simulink model "SMXQ6_600_FOCgains"  (R2026b)
settings: Solver=VariableStepAuto  StopTime=0
model workspace (MAT data in the model file):
  IMax = 10.2
  J = 0.0243
  Ld = 0.0018
  Lq = 0.0018
  Rs = 0.3
  SF = 1
  Ts = 5e-05
  Tsc = 5e-05
libraries: mcbcontrollergainlib x1
settings Model: Creator=Uriel  LastModifiedBy=Uriel

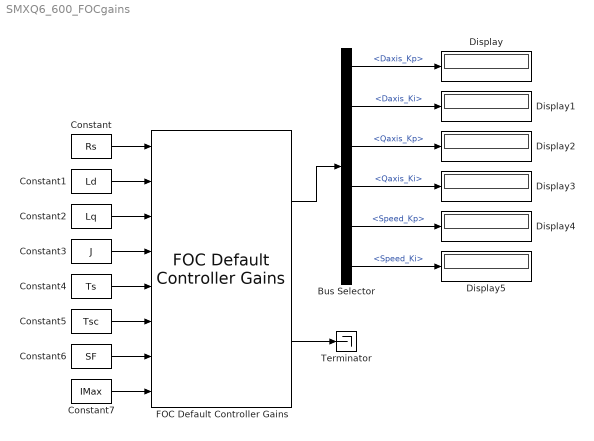
== system SMXQ6_600_FOCgains ==
  Bus Selector : BusSelector  OutputSignals=Daxis_Kp,Daxis_Ki,Qaxis_Kp,Qaxis_Ki,Speed_Kp,Speed_Ki
  Constant : Constant  Value=Rs
  Constant1 : Constant  Value=Ld
  Constant2 : Constant  Value=Lq
  Constant3 : Constant  Value=J
  Constant4 : Constant  Value=Ts
  Constant5 : Constant  Value=Tsc
  Constant6 : Constant  Value=SF
  Constant7 : Constant  Value=IMax
  Display{,1..5} (6 alike) : Display
  FOC Default Controller Gains : mcbcontrollergainlib/FOC Default Controller Gains  ControllerGainType=Empirical method  motorSelection=PMSM  unitType=SI Unit  EnObserver=off  ObsType=Flux Observer (Only for SPMSM)  ObsCutOffFrq=10  outCurrentControlGain=on  outFWCGain=off  outSpeedControlGain=on  externalDelay=off  currentSensorDelay=50e-6  speedSensorDelay=50e-6  speedFilterDelay=0.02
      settings: LibrarySourceBlock=mcblib/Controls/Controllers/FOC Default Controller Gains
  Terminator : Terminator
  wires:
  FOC Default Controller Gains/2 -> Terminator/1
  Constant/1 -> FOC Default Controller Gains/1
  Constant1/1 -> FOC Default Controller Gains/2
  Constant2/1 -> FOC Default Controller Gains/3
  Constant3/1 -> FOC Default Controller Gains/4
  Constant4/1 -> FOC Default Controller Gains/5
  Constant5/1 -> FOC Default Controller Gains/6
  Constant6/1 -> FOC Default Controller Gains/7
  Constant7/1 -> FOC Default Controller Gains/8
  FOC Default Controller Gains/1 -> Bus Selector/1
  Bus Selector/1 -> Display/1  "<Daxis_Kp>"
  Bus Selector/2 -> Display1/1  "<Daxis_Ki>"
  Bus Selector/3 -> Display2/1  "<Qaxis_Kp>"
  Bus Selector/4 -> Display3/1  "<Qaxis_Ki>"
  Bus Selector/5 -> Display4/1  "<Speed_Kp>"
  Bus Selector/6 -> Display5/1  "<Speed_Ki>"
